simulink model "MATLAB"  (R2023a)
settings: Solver=FixedStepAuto  StartTime=0.0  StopTime=inf  FixedStep=0.001  RelTol=1e-3
PreLoadFcn:
  | % 保存原来全局配置，后面关闭模型恢复
  | evalin('base','orig_codegen_folder = Simulink.fileGenControl(''get'',''CodeGenFolder'');');
  | % 设置本模型专属代码输出目录
  | Simulink.fileGenControl('set','CodeGenFolder','D:\HuaweiMoveData\Users\Qw011\Desktop\GitHub\RS\code\E\E_CPU1\ra\fsp\src\MATLAB','CreateDir',true);
libraries: simulink x1
CloseFcn:
  | try
  |     if exist('orig_codegen_folder','var')
  |         Simulink.fileGenControl('set','CodeGenFolder',orig_codegen_folder);
  |         clear orig_codegen_folder;
  |     end
  | catch ME
  |     disp(ME.message);
  | end
settings Model: Creator=Qw011  LastModifiedBy=Qw011
settings OptimizationCC: DefaultParameterBehavior=Inlined  EnhancedBackFolding=on  PassReuseOutputArgsAs=Individual arguments  ZeroExternalMemoryAtStartup=off  ZeroInternalMemoryAtStartup=off  OptimizeBlockOrder=speed  DifferentSizesBufferReuse=on  OptimizationCustomize=off  EfficientTunableParamExpr=on
settings DebuggingCC: ParameterTunabilityLossMsg=error
settings SFSimCC: MATLABDynamicMemAlloc=off
settings RTWCC: Description=Embedded Coder  SystemTargetFile=ert.tlc  TemplateMakefile=ert_default_tmf
settings CodeAppCC: ForceParamTrailComments=on  IgnoreCustomStorageClasses=off  OperatorAnnotations=on  SimulinkDataObjDesc=on  SFDataObjDesc=on  InsertBlockDesc=on
settings ERTTargetCC: TargetLangStandard=C99 (ISO)  InlinedParameterPlacement=NonHierarchical  ERTCustomFileTemplate=example_file_process.tlc

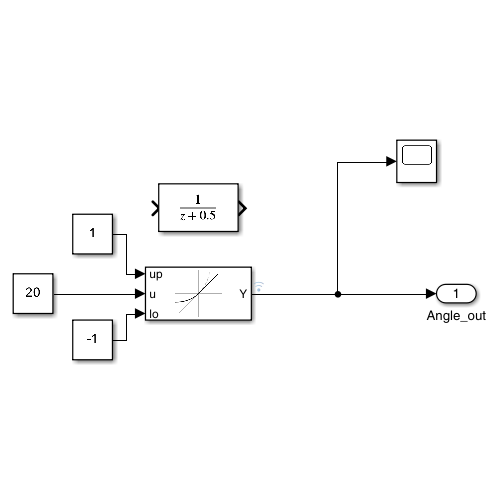
[thumbnail: Simulink's stored preview of the top-level diagram]
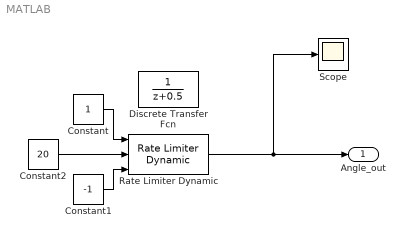
== system MATLAB ==
  Constant : Constant
  Constant1 : Constant  Value=-1
  Constant2 : Constant  Value=20
  Discrete Transfer Fcn : DiscreteTransferFcn
  Rate Limiter Dynamic : simulink/Discontinuities/Rate Limiter Dynamic
  Scope : Scope
  Angle_out : Outport
  wires:
  Constant/1 -> Rate Limiter Dynamic/1
  Constant1/1 -> Rate Limiter Dynamic/3
  Constant2/1 -> Rate Limiter Dynamic/2
  Rate Limiter Dynamic/1 -> Scope/1, Angle_out/1
